simulink model "Plaque_sphere_simulink"  (R2024a)
settings: Solver=VariableStepAuto  StartTime=0.0  StopTime=11  RelTol=1e-3
values from neighbouring files (symbols this model uses):
  A_m = (n_m * K_t * n_g * K_g) / R_m    [Plaque_sphere_code.m]
  B_eq = J_eq / tau    [Plaque_sphere_code.m]
  J_eq = 0.0017728    [Plaque_sphere_code.m]
  K_bb = 5 / 7 * (g * r_arm) / L_plaque    (= 0.647205194805)    [Plaque_sphere_code.m]
undefined symbols (not defined in the file or in its folder): den_a, den_a2, flg_in, K_int, num_a, num_a2
settings Model: Creator=lfgon  LastModifiedBy=labri
settings DataIOCC: ReturnWorkspaceOutputs=off

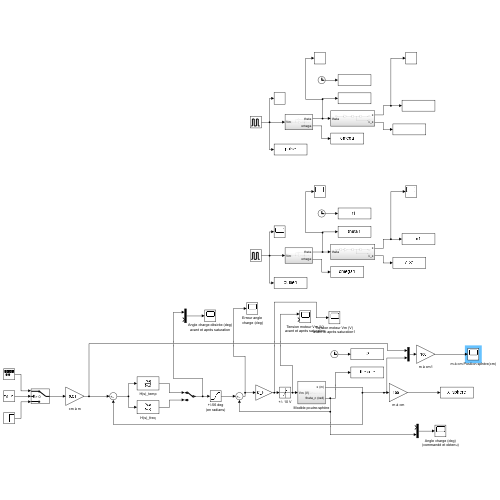
[thumbnail: Simulink's stored preview of the top-level diagram]
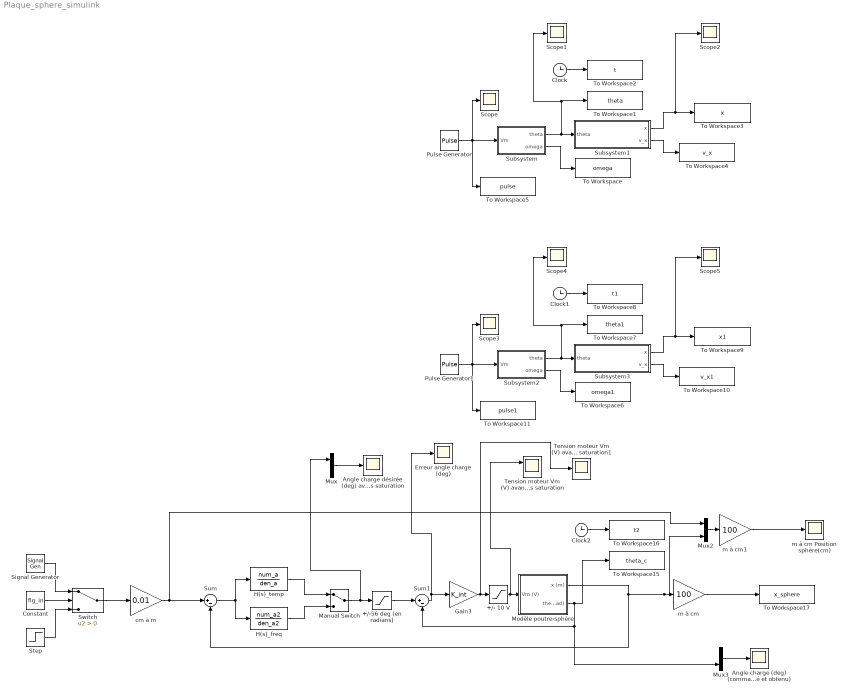
== system Plaque_sphere_simulink ==
  +/- 10 V : Saturate  UpperLimit=10  LowerLimit=-10
  +/-56 deg (en radians) : Saturate  UpperLimit=0.9774  LowerLimit=-0.9774
  Angle charge (deg) (commandé et obtenu) : Scope
  Angle charge désirée (deg) avant et après saturation : Scope
  Clock : Clock
  Clock1 : Clock
  Clock2 : Clock
  Constant : Constant  Value=flg_in
  Erreur angle charge (deg) : Scope
  Gain3 : Gain  Gain=K_int
  H(s)_freq : TransferFcn  Numerator=num_a2  Denominator=den_a2
  H(s)_temp : TransferFcn  Numerator=num_a  Denominator=den_a
  Manual Switch : ManualSwitch
  Modèle poutre-sphère : Subsystem
  Mux : Mux  Inputs=2
  Mux2 : Mux  Inputs=2
  Mux3 : Mux  Inputs=2
  Pulse Generator : DiscretePulseGenerator  PulseType=Time based  Period=6  PulseWidth=50  PhaseDelay=1
  Pulse Generator1 : DiscretePulseGenerator  PulseType=Time based  Period=4  PulseWidth=76  PhaseDelay=1
  Scope{,1..5} (6 alike) : Scope
  Signal Generator : SignalGenerator  WaveForm=square  Units=rad/sec
  Step : Step  After=5  SampleTime=0
  Subsystem : Subsystem
  Subsystem1 : Subsystem
  Subsystem2 : Subsystem
  Subsystem3 : Subsystem
  Sum : Sum  Inputs=|+-
  Sum1 : Sum  Inputs=|+-
  Switch : Switch  Criteria=u2 > Threshold  SaturateOnIntegerOverflow=off  InputSameDT=off
  Tension moteur Vm (V) avant et après saturation : Scope  NumInputPorts=2
  Tension moteur Vm (V) avant et après saturation1 : Scope
  To Workspace : ToWorkspace  VariableName=omega  SampleTime=-1
  To Workspace1 : ToWorkspace  VariableName=theta  SampleTime=-1
  To Workspace10 : ToWorkspace  VariableName=v_x1  SampleTime=-1
  To Workspace11 : ToWorkspace  VariableName=pulse1  SampleTime=-1
  To Workspace15 : ToWorkspace  VariableName=theta_c  SampleTime=-1
  To Workspace16 : ToWorkspace  VariableName=t2  SampleTime=-1
  To Workspace17 : ToWorkspace  VariableName=x_sphere  SampleTime=-1
  To Workspace2 : ToWorkspace  VariableName=t  SampleTime=-1
  To Workspace3 : ToWorkspace  VariableName=x  SampleTime=-1
  To Workspace4 : ToWorkspace  VariableName=v_x  SampleTime=-1
  To Workspace5 : ToWorkspace  VariableName=pulse  SampleTime=-1
  To Workspace6 : ToWorkspace  VariableName=omega1  SampleTime=-1
  To Workspace7 : ToWorkspace  VariableName=theta1  SampleTime=-1
  To Workspace8 : ToWorkspace  VariableName=t1  SampleTime=-1
  To Workspace9 : ToWorkspace  VariableName=x1  SampleTime=-1
  cm à m : Gain  Gain=0.01
  m à cm : Gain  Gain=100
  m à cm Position sphère(cm) : Scope
  m à cm1 : Gain  Gain=100
  wires:
  Clock/1 -> To Workspace2/1
  Subsystem/2(omega) -> To Workspace/1
  Subsystem/1(theta) -> Scope1/1, To Workspace1/1, Subsystem1/1(theta)
  Subsystem1/1(x) -> Scope2/1, To Workspace3/1
  Subsystem1/2(v_x) -> To Workspace4/1
  Pulse Generator/1 -> To Workspace5/1, Scope/1, Subsystem/1(Vm)
  Subsystem2/1(theta) -> Scope4/1, To Workspace7/1, Subsystem3/1(theta)
  Subsystem3/2(v_x) -> To Workspace10/1
  Pulse Generator1/1 -> To Workspace11/1, Scope3/1, Subsystem2/1(Vm)
  Subsystem3/1(x) -> Scope5/1, To Workspace9/1
  Clock1/1 -> To Workspace8/1
  Subsystem2/2(omega) -> To Workspace6/1
  Clock2/1 -> To Workspace16/1
  Sum/1 -> H(s)_freq/1, H(s)_temp/1
  Modèle poutre-sphère/2(theta_c (rad)) -> Mux3/2, Sum1/2, To Workspace15/1
  Sum1/1 -> Gain3/1, Erreur angle charge (deg)/1
  Signal Generator/1 -> Switch/1
  Constant/1 -> Switch/2
  cm à m/1 -> Mux2/1, Sum/1
  m à cm/1 -> To Workspace17/1
  Mux/1 -> Angle charge désirée (deg) avant et après saturation/1
  Step/1 -> Switch/3
  Switch/1 -> cm à m/1
  Modèle poutre-sphère/1(x (m)) -> Mux2/2, m à cm/1, Sum/2
  H(s)_temp/1 -> Manual Switch/1
  H(s)_freq/1 -> Manual Switch/2
  Gain3/1 -> Tension moteur Vm (V) avant et après saturation1/1, +/- 10 V/1
  m à cm1/1 -> m à cm Position sphère(cm)/1
  Mux2/1 -> m à cm1/1
  Mux3/1 -> Angle charge (deg) (commandé et obtenu)/1
  +/- 10 V/1 -> Tension moteur Vm (V) avant et après saturation/1, Modèle poutre-sphère/1(Vm (V))
  Manual Switch/1 -> Mux/1, +/-56 deg (en radians)/1
  +/-56 deg (en radians)/1 -> Sum1/1

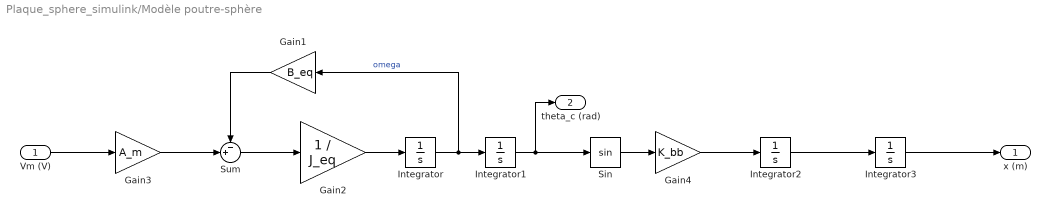
== system Plaque_sphere_simulink/Modèle poutre-sphère ==
  Vm (V) : Inport
  Gain1 : Gain  Gain=B_eq
  Gain2 : Gain  Gain=1 / J_eq
  Gain3 : Gain  Gain=A_m
  Gain4 : Gain  Gain=K_bb
  Integrator{,1..3} (4 alike) : Integrator
  Sin : Trigonometry
  Sum : Sum  Inputs=-+|
  x (m) : Outport
  theta_c (rad) : Outport  Port=2
  wires:
  Sum/1 -> Gain2/1
  Vm (V)/1 -> Gain3/1
  Integrator/1 -> Gain1/1, Integrator1/1  "omega"
  Gain1/1 -> Sum/1
  Gain3/1 -> Sum/2
  Gain2/1 -> Integrator/1
  Integrator3/1 -> x (m)/1
  Integrator2/1 -> Integrator3/1
  Sin/1 -> Gain4/1
  Gain4/1 -> Integrator2/1
  Integrator1/1 -> Sin/1, theta_c (rad)/1

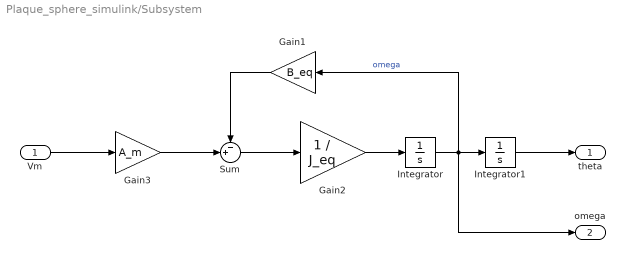
== system Plaque_sphere_simulink/Subsystem ==
  Vm : Inport
  Gain1 : Gain  Gain=B_eq
  Gain2 : Gain  Gain=1 / J_eq
  Gain3 : Gain  Gain=A_m
  Integrator : Integrator
  Integrator1 : Integrator
  Sum : Sum  Inputs=-+|
  theta : Outport
  omega : Outport  Port=2
  wires:
  Sum/1 -> Gain2/1
  Vm/1 -> Gain3/1
  Integrator/1 -> omega/1, Gain1/1, Integrator1/1  "omega"
  Gain1/1 -> Sum/1
  Gain3/1 -> Sum/2
  Gain2/1 -> Integrator/1
  Integrator1/1 -> theta/1

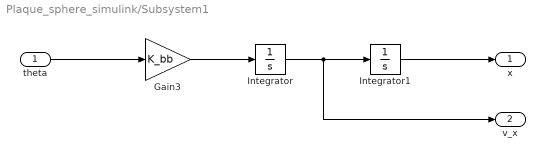
== system Plaque_sphere_simulink/Subsystem1 ==
  theta : Inport
  Gain3 : Gain  Gain=K_bb
  Integrator : Integrator
  Integrator1 : Integrator
  x : Outport
  v_x : Outport  Port=2
  wires:
  Integrator/1 -> v_x/1, Integrator1/1
  Gain3/1 -> Integrator/1
  Integrator1/1 -> x/1
  theta/1 -> Gain3/1

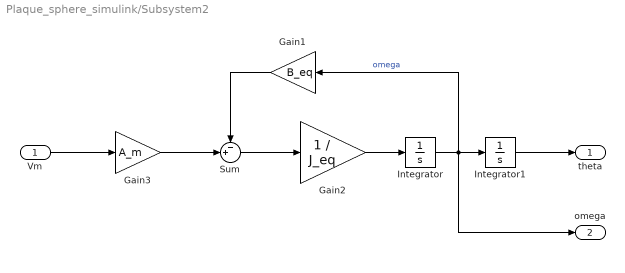
== system Plaque_sphere_simulink/Subsystem2 ==
  Vm : Inport
  Gain1 : Gain  Gain=B_eq
  Gain2 : Gain  Gain=1 / J_eq
  Gain3 : Gain  Gain=A_m
  Integrator : Integrator
  Integrator1 : Integrator
  Sum : Sum  Inputs=-+|
  theta : Outport
  omega : Outport  Port=2
  wires:
  Sum/1 -> Gain2/1
  Vm/1 -> Gain3/1
  Integrator/1 -> omega/1, Gain1/1, Integrator1/1  "omega"
  Gain1/1 -> Sum/1
  Gain3/1 -> Sum/2
  Gain2/1 -> Integrator/1
  Integrator1/1 -> theta/1

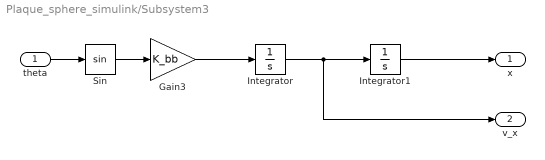
== system Plaque_sphere_simulink/Subsystem3 ==
  theta : Inport
  Gain3 : Gain  Gain=K_bb
  Integrator : Integrator
  Integrator1 : Integrator
  Sin : Trigonometry
  x : Outport
  v_x : Outport  Port=2
  wires:
  Integrator/1 -> v_x/1, Integrator1/1
  Gain3/1 -> Integrator/1
  Integrator1/1 -> x/1
  theta/1 -> Sin/1
  Sin/1 -> Gain3/1
